simulink model "TPS_DAB_Avik"  (R2026b)
settings: Solver=VariableStepAuto  StopTime=3e-3
values from neighbouring files (symbols this model uses):
  del_t = D1*T_hs    (= 3.125e-06)    [calib_params.m]
  R_load = 40    [calib_params.m]
  T_hs = T_s/2    (= 1.25e-05)    [calib_params.m]
  T_s = 1/f_sw    (= 2.5e-05)    [calib_params.m]
libraries: nesl_utility x16, ee_lib x16, fl_lib x14
settings Model: Creator=EV5_1  LastModifiedBy=avikd
settings SimscapeCC: SimscapeLogType=all  SimscapeNominalValues="[{\"value\":\"1\",\"unit\":\"A\"},{\"value\":\"1\",\"unit\":\"bar\"},{\"value\":\"1\",\"unit\":\"cm^2\"},{\"value\":\"1\",\"unit\":\"cm^3/s\"},{\"value\":\"1\",\"unit\":\"kJ/kg\"},{\"value\":\"1\",\"unit\":\"kW\"},{\"value\":\"1\",\"unit\":\"l\"},{\"value\":\"1\",\"unit\":\"N\"},{\"value\":\"1\",\"unit\":\"N*m\"},{\"value\":\"1\",\"unit\":\"V\"},{\"value\":\"0.001\",\"unit\":\"Wb\"}]"  SimscapeUseEnergyAccounting=off

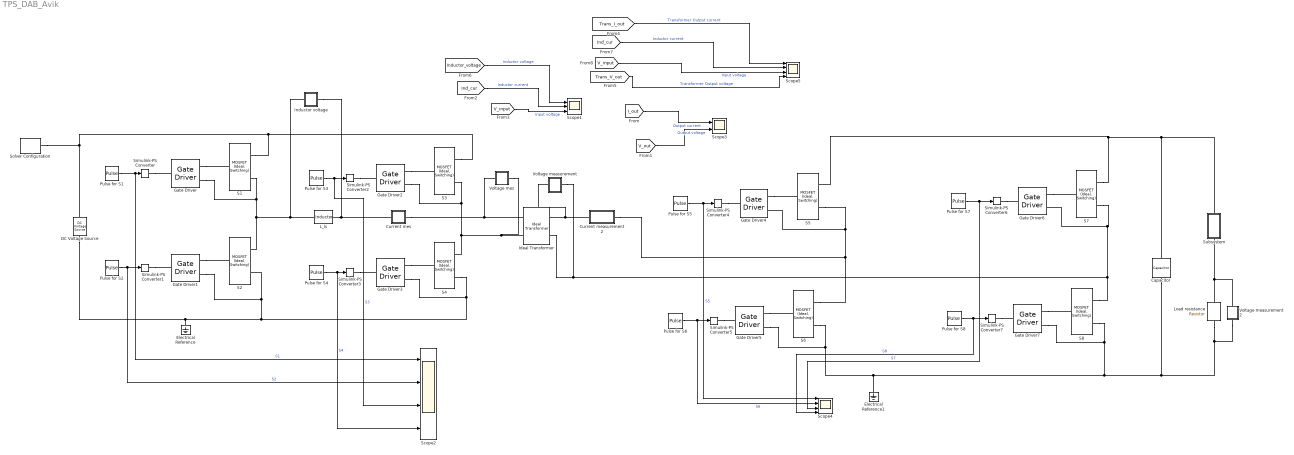
== system TPS_DAB_Avik ==
  Capacitor : fl_lib/Electrical/Electrical Elements/Capacitor  c=Cout uF  r=Cout_ESR Ohm  g=0 1/Ohm  i_specify=off  i_priority=None  i=0 A  i_nominal_specify=off  i_nominal_value=1  i_nominal_unit=A  v_specify=off  v_priority=None  v=0 V  v_nominal_specify=off  v_nominal_value=1  v_nominal_unit=V  vc_specify=off  vc_priority=High  vc=0 V  vc_nominal_specify=off  vc_nominal_value=1  vc_nominal_unit=V
  Current measurement 2 : Subsystem
  Current mes : Subsystem
  DC Voltage Source : fl_lib/Electrical/Electrical Sources/DC Voltage Source  v0=100 V
  Electrical Reference : fl_lib/Electrical/Electrical Elements/Electrical Reference
  Electrical Reference1 : fl_lib/Electrical/Electrical Elements/Electrical Reference
  Gate Driver{,1..7} (8 alike) : ee_lib/Semiconductors & Converters/Gate Driver  port_option=ee.enum.controlport.ps  uHigh=2.0 V  uLow=0.8 V  uHighValue=0.7  uLowValue=0.3  vHigh=15 V  vLow=0 V  tHigh=50 ns  tLow=50 ns  parameterization=ee.enum.semiconductors.gateDriverParam.outputImpedance  rHigh=2 Ohm  rLow=2 Ohm  tRise=20 ns  tFall=20 ns  cLoad=10 nF  ZonTime_specify=off  ZonTime_priority=None  ZonTime=0 s  ZoffTime_specify=off  ZoffTime_priority=None  ZoffTime=0 s
  Ideal Transformer : fl_lib/Electrical/Electrical Elements/Ideal Transformer  n=2  i1_specify=off  i1_priority=None  i1=0 A  i1_nominal_specify=off  i1_nominal_value=1  i1_nominal_unit=A  v1_specify=off  v1_priority=None  v1=0 V  v1_nominal_specify=off  v1_nominal_value=1  v1_nominal_unit=V  i2_specify=off  i2_priority=None  i2=0 A  i2_nominal_specify=off  i2_nominal_value=1  i2_nominal_unit=A  v2_specify=off  v2_priority=None  v2=0 V  v2_nominal_specify=off  v2_nominal_value=1  v2_nominal_unit=V
  Inductor voltage : Subsystem
  L_ls : fl_lib/Electrical/Electrical Elements/Inductor  l=L_ls H  r=L_ls_ESR Ohm  g=1e-9 1/Ohm  i_specify=off  i_priority=None  i=0 A  i_nominal_specify=off  i_nominal_value=1  i_nominal_unit=A  v_specify=off  v_priority=None  v=0 V  v_nominal_specify=off  v_nominal_value=1  v_nominal_unit=V  i_L_specify=off  i_L_priority=High  i_L=0 A  i_L_nominal_specify=off  i_L_nominal_value=1  i_L_nominal_unit=A
  Load resistance : fl_lib/Electrical/Electrical Elements/Resistor  R=R_load Ohm  i_specify=off  i_priority=None  i=0 A  i_nominal_specify=off  i_nominal_value=1  i_nominal_unit=A  v_specify=off  v_priority=None  v=0 V  v_nominal_specify=off  v_nominal_value=1  v_nominal_unit=V
  Pulse for S1 : DiscretePulseGenerator  PulseType=Time based  Period=T_s  PulseWidth=50
  Pulse for S2 : DiscretePulseGenerator  PulseType=Time based  Period=T_s  PulseWidth=50  PhaseDelay=T_hs
  Pulse for S3 : DiscretePulseGenerator  PulseType=Time based  Period=T_s  PulseWidth=50  PhaseDelay=T_hs
  Pulse for S4 : DiscretePulseGenerator  PulseType=Time based  Period=T_s  PulseWidth=50
  Pulse for S5 : DiscretePulseGenerator  PulseType=Time based  Period=T_s  PulseWidth=50  PhaseDelay=del_t
  Pulse for S6 : DiscretePulseGenerator  PulseType=Time based  Period=T_s  PulseWidth=50  PhaseDelay=T_hs+del_t
  Pulse for S7 : DiscretePulseGenerator  PulseType=Time based  Period=T_s  PulseWidth=50  PhaseDelay=T_hs+del_t
  Pulse for S8 : DiscretePulseGenerator  PulseType=Time based  Period=T_s  PulseWidth=50  PhaseDelay=del_t
  S{1..8} (8 alike) : ee_lib/Semiconductors & Converters/MOSFET (Ideal, Switching)  port_option=ee.enum.controlport.elec  Rds=0.01 Ohm  Goff=1e-6 1/Ohm  Vth=2 V  diode_param=ee.enum.semiconductors.protectionDiode.nodynamics  diode_Vf=0.8 V  diode_Ron=0.001 Ohm  diode_Goff=1e-5 1/Ohm  diode_C=50e-9 F  diode_iRM=-235 A  diode_iF=300 A  diode_idot=-50 A/us  diode_trr_param=ee.enum.converters.diodeReverseParam.trr_factor  diode_trr_factor=3  diode_trr=15 us  diode_Qrr=1500 s*uA  ids_specify=off  ids_priority=None  ids=0 A  ids_nominal_specify=off  ids_nominal_value=1  ids_nominal_unit=A  vds_specify=off  vds_priority=None  vds=0 V  vds_nominal_specify=off  vds_nominal_value=1  vds_nominal_unit=V  vgs_specify=off  vgs_priority=None  vgs=0 V  vgs_nominal_specify=off  vgs_nominal_value=1  vgs_nominal_unit=V  thermal_loss_option=ee.enum.converters.thermalLossOption.constantvalues  Von_data=[0, 1.8, 3.2, 6, 10, 16; 0, 2, 5.5, 9.5, 15, 25] V  Tj=[298.15, 448.15] K  Iout_data=[0, 20, 40, 60, 80, 100] A  tabulateWithVds=false  Eon_data=[0, 55.04, 124.57, 235.53, 362.12; 0, 71.25, 161.25, 304.88, 468.75] * 1e-6 J  Eoff_data=[0, 18, 30, 56.1, 76.5; 0, 22.5, 37.5, 70.13, 95.63] * 1e-6 J  Eon_data_3D=[zeros(2, 5, 3)] J  Eoff_data_3D=[zeros(2, 5, 3)] J  Tj_loss=[298.15, 448.15] K  Iout_data_loss=[0, 10, 20, 30, 40] A  Vds_loss=[0, 150, 300] V  Eon_scalar=22.86e-3 J  Eoff_scalar=17.14e-3 J  Voff=300 V  Iout_scalar=600 A  useCurrentFromPreviousCycle=false  currentMeasDelay=0 s  useVoltageFromPreviousCycle=false  voltageMeasDelay=0 s  diodeModelType=ee.enum.converters.diodeModelType.pwl  diodeTableType=ee.enum.diode.tableType.IfMat  diode_ReverseIVType=ee.enum.diode.diodeReverseIV.constant  diode_IfMat=[.07, .12, .19, 1.75, 4.24, 7.32, 11.2; .16, .3, .72, 2.14, 4.02, 6.35, 9.12] A  diode_VfMat=[.9, 1.15, 1.25, 1.5, 1.75, 2.17, 2.6, 2.85; .58, .68, .75, 1.1, 1.38, 1.77, 2.27, 2.7] V  diode_TjVec=[25, 125] degC  diode_VfVec=[.5, .7, .9, 1.3, 1.7, 2.1, 2.5] V  diode_IfVec=[.1, .2, .5, 1, 2, 4, 7, 10] A  diode_IrMat=[1e-06, 2e-06, 5e-06, 1e-05, 2.5e-05, 5e-05, .0001; 2e-06, 5e-06, 1e-05, 4e-05, 8e-05, .0002, .0005] A  diode_VrMat=[10, 100, 200, 250, 300, 325, 350; 10, 70, 160, 220, 270, 300, 320] V  diode_VrVec=[10, 20, 40, 50, 70, 80, 100] V  diode_IrVec=[1e-06, 2e-06, 5e-06, 1e-05, 2e-05, 5e-05, .0001] A  diode_Vr=-600 V  diode_Ls=150 nH  diode_Erec=0.03 J  diode_rec_loss_model=ee.enum.diode.reverseRecoveryModelTabulateUpTo3D.fixed  diode_ErecVal=0 J  diode_scaleWithIandV=true  diode_ErecMat=zeros(2, 3) J  diodeErecMat3D=zeros(2, 3, 2) J  diode_TjrecVec=[298.15, 398.15] K  diode_IfrecVec=[.1, 1, 10] A  diodeVrecVec=[0, 100] V  diode_IrecVal=10 A  diode_VrecVal=10 V  diode_tFilter=1 / 1000 / 100 s  separateThermalPortForDiode=false  thermal_network_parameterization=ee.enum.thermalNetworkTopology.external  Rth=[.03, .2] K/W  Rth_Cauer=[.03, .1, .2] K/W  Rth_Foster=[.08, .14, .22, .16] K/W  thermal_mass_parameterization=ee.enum.thermalNetwork.timeconstant  thermal_mass=[3, 25] J/K  thermal_mass_Cauer=[3, 10, 25] J/K  thermal_mass_Foster=[.001, .005, .05, .5] J/K  thermal_time_constant=[.1, 5] s  thermal_time_constant_Cauer=[.1, 1, 5] s  thermal_time_constant_Foster=[7e-05, .0007, .01, .08] s  thermal_mass_initial_temperatures=[25, 25] degC  thermal_mass_initial_temperatures_Cauer=[25, 25, 25] degC  junction_thermal_mass=0.1 J/K  Tvec_initial_Foster=[25, 25, 25, 25] degC  RthDiode=[.03, .2] K/W  RthCauerDiode=[.03, .1, .2] K/W  RthFosterDiode=[.03, .2] K/W  thermalMassDiode=[3, 25] J/K  thermalMassCauerDiode=[3, 10, 25] J/K  thermalMassFosterDiode=[33, 50] J/K  thermalTauDiode=[.1, 5] s  thermalTauCauerDiode=[.1, 1, 5] s  thermalTauFosterDiode=[1, 10] s  thermalMassInitTempDiode=[25, 25] degC  thermalMassInitTempCauerDiode=[25, 25, 25] degC  junctionthermalMassDiode=0.1 J/K  TVecInitialFosterDiode=[25, 25, 25, 25] degC  no_thermal_network=ee.enum.enable.no  mosfet_junction_temperature_specify=off  mosfet_junction_temperature_priority=None  mosfet_junction_temperature=25 degC  mosfet_junction_temperature_nominal_specify=off  mosfet_junction_temperature_nominal_value=1  mosfet_junction_temperature_nominal_unit=degC  diode_junction_temperature_specify=off  diode_junction_temperature_priority=None  diode_junction_temperature=25 degC  diode_junction_temperature_nominal_specify=off  diode_junction_temperature_nominal_value=1  diode_junction_temperature_nominal_unit=degC  Qj_specify=off  Qj_priority=None  Qj=0 W  Qj_nominal_specify=off  Qj_nominal_value=1  Qj_nominal_unit=W  accumulatedSwitchingLosses_specify=off  accumulatedSwitchingLosses_priority=None  accumulatedSwitchingLosses=0 J
  Scope1 : Scope  NumInputPorts=3
      settings: ActiveDisplayYMinimum=-462.98345997491094  ActiveDisplayYMaximum=426.570481445315
  Scope2 : Scope  NumInputPorts=4
      settings: ActiveDisplayYMinimum=-0.12499999999999997  ActiveDisplayYMaximum=1.125  DataLoggingVariableName=ScopeData2
  Scope3 : Scope  NumInputPorts=2
      settings: ActiveDisplayYMinimum=-4.0372091768871385  ActiveDisplayYMaximum=8.9618480770754481  DataLoggingVariableName=ScopeData3
  Scope4 : Scope  NumInputPorts=4
      settings: ActiveDisplayYMinimum=-0.12499999999999997  ActiveDisplayYMaximum=1.125  DataLoggingVariableName=ScopeData4
  Scope5 : Scope  NumInputPorts=4
      settings: ActiveDisplayYMinimum=-6.1323676856084512  ActiveDisplayYMaximum=12.915642777328962  DataLoggingVariableName=ScopeData5
  Simulink-PS Converter{,1..7} (8 alike) : nesl_utility/Simulink-PS Converter  PhysicalDomain=network_engine_domain  SubClassName=ps_input  LeftPortType=input  RightPortType=output  PseudoPeriodic=off  Frequencies=[]  NoiseDistribution=none  NoiseParameters=[]  Unit=1  AffineConversion=off  FilteringAndDerivatives=provide  SimscapeFilterOrder=1  InputFilterTimeConstant=0.001  UdotUserProvided=0
  Solver Configuration : nesl_utility/Solver Configuration  PhysicalDomain=network_engine_domain  SubClassName=solver  LeftPortType=input  RightPortType=generic  Tones=[]  Harmonics=[]  SimulateNoise=off  Profile=off  UseLocalSampling=off  EnableSwitchedLinearOptims=on  FrequencyDomain=off  UseCCode=off  RelTol=0.001  AbsTol=0.001  MinStep=1e-09  ToWorkspace=off  RevertToSquareIcSolve=off  NumHomotopyIterations=100  PhasorMode=off  PhasorModeNumHarmonics=1  ConsistencySolver=NEWTON_XTOL_AFTER_FTOL  CanonicalOrdering=CANONICAL  OptimizeIntermediates=OPTIMIZED  MulticoreSolverChoice=BACKWARD_EULER  IndexReductionMethod=DerivativeReplacement  DoDC=off  ResidualTolerance=1e-09  ConsistencyTolSource=GLOBAL  ConsistencyAbsTol=0.001  ConsistencyRelTol=0.001  ConsistencyTolFactor=0.001  UseLocalSolver=on  LocalSolverChoice=NE_BACKWARD_EULER_ADVANCER  ResolveIndetEquations=on  FunctionEvalNumThread=1  LocalSolverSampleTime=1e-7  DoFixedCost=off  MaxNonlinIter=3  MaxModeIter=2  ComputeImpulses=off  ImpulseIterations=2  LinearAlgebra=auto  LinearAlgebraNumThread=0  EquationFormulation=NE_TIME_EF  DelaysMemoryBudget=1024  AutomaticFiltering=on  FilteringTimeConstant=0.001  PartitionStorageMethod=AS_NEEDED  PartitionMemoryBudget=1024  PartitionMethod=BALANCED  MultibodyUseLocalSolver=off  MultibodyLocalSolverChoice=ODE1  MultibodyLocalSolverSampleTime=0.001
  Subsystem : Subsystem
  Voltage measurement : Subsystem
  Voltage measurement 2 : Subsystem
  Voltage mes : Subsystem
  wires:
  Pulse for S1/1 -> Scope2/1, Simulink-PS Converter/1  "S1"
  Pulse for S2/1 -> Scope2/2, Simulink-PS Converter1/1  "S2"
  Pulse for S4/1 -> Scope2/4, Simulink-PS Converter3/1  "S4"
  Pulse for S3/1 -> Scope2/3, Simulink-PS Converter2/1  "S3"
  [V_input] -> Scope1/3  "Input voltage"
  Pulse for S5/1 -> Scope4/1, Simulink-PS Converter4/1  "S5"
  Pulse for S6/1 -> Scope4/2, Simulink-PS Converter5/1  "S6"
  Pulse for S7/1 -> Scope4/3, Simulink-PS Converter6/1  "S7"
  Pulse for S8/1 -> Scope4/4, Simulink-PS Converter7/1  "S8"
  [I_out] -> Scope3/1  "Output current"
  [V_out] -> Scope3/2  "Output voltage"
  [Ind_cur] -> Scope1/2  "Inductor current"
  [Trans_V_out] -> Scope5/4  "Transformer Output voltage"
  [Trans_I_out] -> Scope5/1  "Transformer Output current"
  [Inductor_voltage] -> Scope1/1  "Inductor voltage"
  [Ind_cur] -> Scope5/2  "Inductor current"
  [V_input] -> Scope5/3  "Input voltage"
  connections:
  Gate Driver/RConn1 -- S1/LConn1
  Simulink-PS Converter/RConn1 -- Gate Driver/LConn1
  Gate Driver1/RConn1 -- S2/LConn1
  Simulink-PS Converter1/RConn1 -- Gate Driver1/LConn1
  S1/RConn2 -- Gate Driver/RConn2 -- Inductor voltage/LConn1 -- L_ls/LConn1 -- S2/RConn1
  DC Voltage Source/LConn1 -- Solver Configuration/RConn1 -- S3/RConn1 -- S1/RConn1
  DC Voltage Source/RConn1 -- Electrical Reference/LConn1 -- Gate Driver3/RConn2 -- S4/RConn2 -- Gate Driver1/RConn2 -- S2/RConn2
  S3/RConn2 -- Gate Driver2/RConn2 -- Voltage mes/RConn1 -- Ideal Transformer/LConn2 -- S4/RConn1
  Simulink-PS Converter3/RConn1 -- Gate Driver3/LConn1
  Gate Driver2/RConn1 -- S3/LConn1
  Gate Driver3/RConn1 -- S4/LConn1
  Simulink-PS Converter2/RConn1 -- Gate Driver2/LConn1
  Simulink-PS Converter4/RConn1 -- Gate Driver4/LConn1
  Gate Driver4/RConn1 -- S5/LConn1
  Simulink-PS Converter5/RConn1 -- Gate Driver5/LConn1
  Gate Driver5/RConn1 -- S6/LConn1
  Gate Driver6/RConn1 -- S7/LConn1
  Gate Driver7/RConn1 -- S8/LConn1
  Simulink-PS Converter6/RConn1 -- Gate Driver6/LConn1
  Simulink-PS Converter7/RConn1 -- Gate Driver7/LConn1
  S5/RConn2 -- Current measurement 2/RConn1 -- S6/RConn1 -- Gate Driver4/RConn2
  S7/RConn2 -- Ideal Transformer/RConn2 -- Voltage measurement/RConn1 -- S8/RConn1 -- Gate Driver6/RConn2
  S7/RConn1 -- Capacitor/LConn1 -- Subsystem/LConn1 -- S5/RConn1
  S6/RConn2 -- Electrical Reference1/LConn1 -- Voltage measurement 2/RConn1 -- Load resistance/RConn1 -- Capacitor/RConn1 -- Gate Driver7/RConn2 -- S8/RConn2 -- Gate Driver5/RConn2
  Subsystem/RConn1 -- Voltage measurement 2/LConn1 -- Load resistance/LConn1
  L_ls/RConn1 -- Inductor voltage/RConn1 -- Current mes/LConn1
  Current mes/RConn1 -- Voltage mes/LConn1 -- Ideal Transformer/LConn1
  Current measurement 2/LConn1 -- Ideal Transformer/RConn1 -- Voltage measurement/LConn1

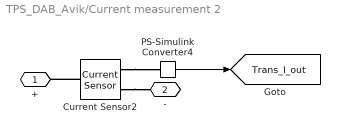
== system TPS_DAB_Avik/Current measurement 2 ==
  Current Sensor2 : fl_lib/Electrical/Electrical Sensors/Current Sensor
  PS-Simulink Converter4 : nesl_utility/PS-Simulink Converter  PhysicalDomain=network_engine_domain  SubClassName=ps_output  LeftPortType=input  RightPortType=output  PseudoPeriodic=off  Frequencies=[]  VectorFormat=inherit  Unit=inherit  AffineConversion=off
  + : PMIOPort  Side=Left
  - : PMIOPort  Port=2  Side=Right
  tag scope: Trans_I_out=global
  wires:
  PS-Simulink Converter4/1 -> [Trans_I_out]
  connections:
  Current Sensor2/RConn1 -- PS-Simulink Converter4/LConn1
  Current Sensor2/RConn2 -- -/RConn1
  Current Sensor2/LConn1 -- +/RConn1

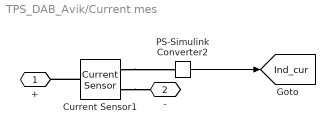
== system TPS_DAB_Avik/Current mes ==
  Current Sensor1 : fl_lib/Electrical/Electrical Sensors/Current Sensor
  PS-Simulink Converter2 : nesl_utility/PS-Simulink Converter  PhysicalDomain=network_engine_domain  SubClassName=ps_output  LeftPortType=input  RightPortType=output  PseudoPeriodic=off  Frequencies=[]  VectorFormat=inherit  Unit=inherit  AffineConversion=off
  + : PMIOPort  Side=Left
  - : PMIOPort  Port=2  Side=Right
  tag scope: Ind_cur=global
  wires:
  PS-Simulink Converter2/1 -> [Ind_cur]
  connections:
  Current Sensor1/RConn1 -- PS-Simulink Converter2/LConn1
  Current Sensor1/LConn1 -- +/RConn1
  Current Sensor1/RConn2 -- -/RConn1

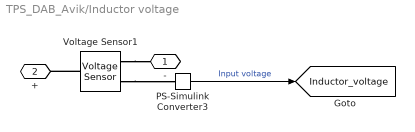
== system TPS_DAB_Avik/Inductor voltage ==
  PS-Simulink Converter3 : nesl_utility/PS-Simulink Converter  PhysicalDomain=network_engine_domain  SubClassName=ps_output  LeftPortType=input  RightPortType=output  PseudoPeriodic=off  Frequencies=[]  VectorFormat=inherit  Unit=inherit  AffineConversion=off
  Voltage Sensor1 : fl_lib/Electrical/Electrical Sensors/Voltage Sensor
  - : PMIOPort  Side=Right
  + : PMIOPort  Port=2  Side=Left
  tag scope: Inductor_voltage=global
  wires:
  PS-Simulink Converter3/1 -> [Inductor_voltage]  "Input voltage"
  connections:
  Voltage Sensor1/RConn1 -- PS-Simulink Converter3/LConn1
  Voltage Sensor1/RConn2 -- -/RConn1
  Voltage Sensor1/LConn1 -- +/RConn1

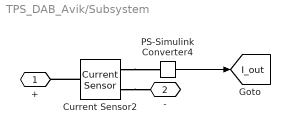
== system TPS_DAB_Avik/Subsystem ==
  Current Sensor2 : fl_lib/Electrical/Electrical Sensors/Current Sensor
  PS-Simulink Converter4 : nesl_utility/PS-Simulink Converter  PhysicalDomain=network_engine_domain  SubClassName=ps_output  LeftPortType=input  RightPortType=output  PseudoPeriodic=off  Frequencies=[]  VectorFormat=inherit  Unit=inherit  AffineConversion=off
  + : PMIOPort  Side=Left
  - : PMIOPort  Port=2  Side=Right
  tag scope: I_out=global
  wires:
  PS-Simulink Converter4/1 -> [I_out]
  connections:
  Current Sensor2/RConn1 -- PS-Simulink Converter4/LConn1
  Current Sensor2/RConn2 -- -/RConn1
  Current Sensor2/LConn1 -- +/RConn1

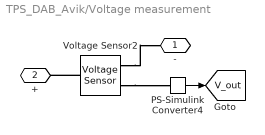
== system TPS_DAB_Avik/Voltage measurement ==
  PS-Simulink Converter4 : nesl_utility/PS-Simulink Converter  PhysicalDomain=network_engine_domain  SubClassName=ps_output  LeftPortType=input  RightPortType=output  PseudoPeriodic=off  Frequencies=[]  VectorFormat=inherit  Unit=inherit  AffineConversion=off
  Voltage Sensor2 : fl_lib/Electrical/Electrical Sensors/Voltage Sensor
  - : PMIOPort  Side=Right
  + : PMIOPort  Port=2  Side=Left
  tag scope: V_out=global
  wires:
  PS-Simulink Converter4/1 -> [V_out]
  connections:
  Voltage Sensor2/RConn1 -- PS-Simulink Converter4/LConn1
  Voltage Sensor2/RConn2 -- -/RConn1
  Voltage Sensor2/LConn1 -- +/RConn1

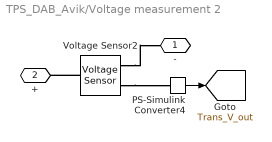
== system TPS_DAB_Avik/Voltage measurement 2 ==
  PS-Simulink Converter4 : nesl_utility/PS-Simulink Converter  PhysicalDomain=network_engine_domain  SubClassName=ps_output  LeftPortType=input  RightPortType=output  PseudoPeriodic=off  Frequencies=[]  VectorFormat=inherit  Unit=inherit  AffineConversion=off
  Voltage Sensor2 : fl_lib/Electrical/Electrical Sensors/Voltage Sensor
  - : PMIOPort  Side=Right
  + : PMIOPort  Port=2  Side=Left
  tag scope: Trans_V_out=global
  wires:
  PS-Simulink Converter4/1 -> [Trans_V_out]
  connections:
  Voltage Sensor2/RConn1 -- PS-Simulink Converter4/LConn1
  Voltage Sensor2/RConn2 -- -/RConn1
  Voltage Sensor2/LConn1 -- +/RConn1

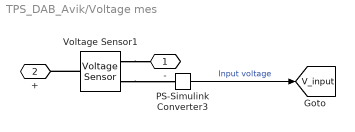
== system TPS_DAB_Avik/Voltage mes ==
  PS-Simulink Converter3 : nesl_utility/PS-Simulink Converter  PhysicalDomain=network_engine_domain  SubClassName=ps_output  LeftPortType=input  RightPortType=output  PseudoPeriodic=off  Frequencies=[]  VectorFormat=inherit  Unit=inherit  AffineConversion=off
  Voltage Sensor1 : fl_lib/Electrical/Electrical Sensors/Voltage Sensor
  - : PMIOPort  Side=Right
  + : PMIOPort  Port=2  Side=Left
  tag scope: V_input=global
  wires:
  PS-Simulink Converter3/1 -> [V_input]  "Input voltage"
  connections:
  Voltage Sensor1/RConn1 -- PS-Simulink Converter3/LConn1
  Voltage Sensor1/RConn2 -- -/RConn1
  Voltage Sensor1/LConn1 -- +/RConn1
